simulink model "FOC_Control"  (R2024b)
settings: Solver=ode4  StartTime=0.0  StopTime=0.5  FixedStep=Ts/10  RelTol=1e-3
InitFcn:
  | foc_param;
values from neighbouring files (symbols this model uses):
  Iq_max = cast(Iq_max, FOC_dtype)    [foc_param.m]
  Ki_dq = make_foc_parameter(Ki_dq_val, FOC_dtype, 'Id/Iq current PI integral gain',     'V/(A*s)')    [foc_param.m]
  Ki_w = make_foc_parameter(Ki_w_val,  FOC_dtype, 'Speed PI integral gain',             'A/rad')    [foc_param.m]
  Kp_dq = make_foc_parameter(Kp_dq_val, FOC_dtype, 'Id/Iq current PI proportional gain', 'V/A')    [foc_param.m]
  Kp_w = make_foc_parameter(Kp_w_val,  FOC_dtype, 'Speed PI proportional gain',         'A/(rad/s)')    [foc_param.m]
  Spd_ref_tau = Kp_w_val/Ki_w_val    [foc_param.m]
  Ts = 1/20000    (= 5e-05)    [foc_param.m]
  Vmax = cast(Vmax,   FOC_dtype)    [foc_param.m]
undefined symbols (not defined in the file or in its folder): DiscIntNeverNeededParam
settings Model: Creator=BitCore  LastModifiedBy=BitCore
settings OptimizationCC: DefaultParameterBehavior=Inlined  EnhancedBackFolding=on  PassReuseOutputArgsAs=Individual arguments  ZeroExternalMemoryAtStartup=off  ZeroInternalMemoryAtStartup=off  OptimizeBlockOrder=speed  DifferentSizesBufferReuse=on  OptimizationCustomize=off  EfficientTunableParamExpr=on
settings DebuggingCC: ParameterTunabilityLossMsg=error
settings HardwareCC: ProdBitPerInt=16  ProdBitPerPointer=16  ProdBitPerSizeT=16  ProdBitPerPtrDiffT=16  ProdLargestAtomicFloat=None  ProdWordSize=16  ProdHWDeviceType=STMicroelectronics->ST10/Super10  TargetBitPerPointer=64  TargetBitPerSizeT=64  TargetBitPerPtrDiffT=64  TargetLongLongMode=on  TargetIntDivRoundTo=Zero  TargetEndianess=LittleEndian  TargetWordSize=64  TargetHWDeviceType=MATLAB Host  ProdEqTarget=off
settings SFSimCC: MATLABDynamicMemAlloc=off
settings RTWCC: Description=Embedded Coder (host-based shared library target)  SystemTargetFile=ert_shrlib.tlc  TemplateMakefile=ert_default_tmf
settings CodeAppCC: ForceParamTrailComments=on  IgnoreCustomStorageClasses=off  OperatorAnnotations=on  SimulinkDataObjDesc=on  SFDataObjDesc=on  InsertBlockDesc=on
settings STFCustomTargetCC: TargetLangStandard=C99 (ISO)  MultiwordLength=256  GenerateSampleERTMain=on  ParMdlRefBuildCompliant=on  CompOptLevelCompliant=on  CombineOutputUpdateFcns=on  ERTCustomFileBanners=on  SupportContinuousTime=off  SupportNonInlinedSFcns=off  RemoveResetFunc=on  MATLABClassNameForMDSCustomization=Simulink.SoftwareTarget.ERTCustomization  ModelStepFunctionPrototypeControlCompliant=on  UseToolchainInfoCompliant=on  SystemTargetFile=ert_shrlib.tlc
settings ERTTargetCC: TargetLangStandard=C99 (ISO)  GenerateSampleERTMain=on  ConcurrentExecutionCompliant=off  CPPClassGenCompliant=off  ERTCustomFileTemplate=example_file_process.tlc

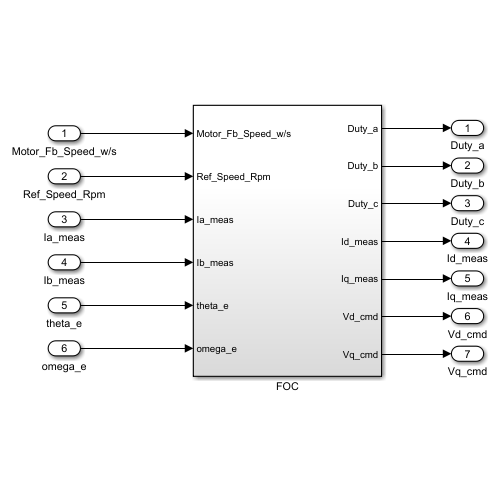
[thumbnail: Simulink's stored preview of the top-level diagram]
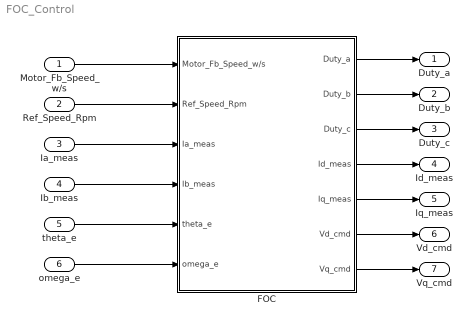
== system FOC_Control ==
  Motor_Fb_Speed_w/s : Inport
  Ref_Speed_Rpm : Inport  Port=2
  Ia_meas : Inport  Port=3
  Ib_meas : Inport  Port=4
  theta_e : Inport  Port=5
  omega_e : Inport  Port=6
  FOC : Subsystem
  Duty_a : Outport
  Duty_b : Outport  Port=2
  Duty_c : Outport  Port=3
  Id_meas : Outport  Port=4
  Iq_meas : Outport  Port=5
  Vd_cmd : Outport  Port=6
  Vq_cmd : Outport  Port=7
  wires:
  Motor_Fb_Speed_w/s/1 -> FOC/1(Motor_Fb_Speed_w/s)
  Ref_Speed_Rpm/1 -> FOC/2(Ref_Speed_Rpm)
  Ia_meas/1 -> FOC/3(Ia_meas)
  Ib_meas/1 -> FOC/4(Ib_meas)
  theta_e/1 -> FOC/5(theta_e)
  omega_e/1 -> FOC/6(omega_e)
  FOC/1(Duty_a) -> Duty_a/1
  FOC/2(Duty_b) -> Duty_b/1
  FOC/3(Duty_c) -> Duty_c/1
  FOC/4(Id_meas) -> Id_meas/1
  FOC/5(Iq_meas) -> Iq_meas/1
  FOC/6(Vd_cmd) -> Vd_cmd/1
  FOC/7(Vq_cmd) -> Vq_cmd/1

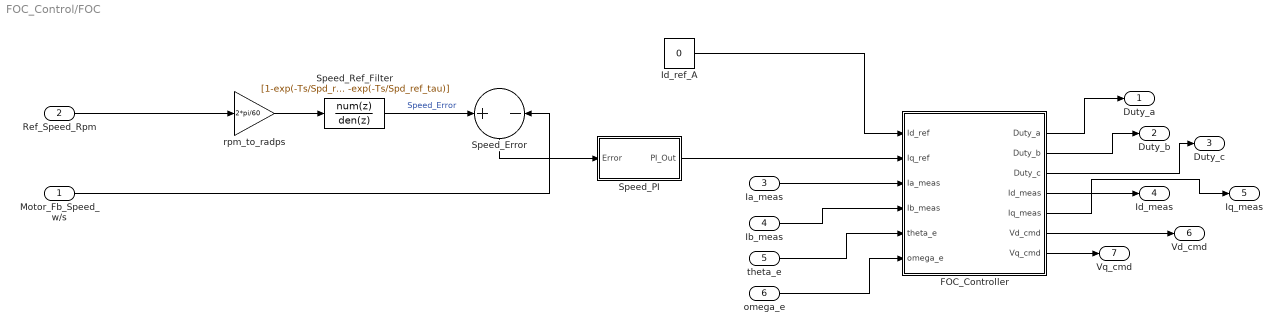
== system FOC_Control/FOC ==
  Motor_Fb_Speed_w/s : Inport
  Ref_Speed_Rpm : Inport  Port=2
  Ia_meas : Inport  Port=3
  Ib_meas : Inport  Port=4
  theta_e : Inport  Port=5
  omega_e : Inport  Port=6
  FOC_Controller : Subsystem
  Id_ref_A : Constant  Value=0
  Speed_Error : Sum  Inputs=+-
  Speed_PI : Subsystem
  Speed_Ref_Filter : DiscreteTransferFcn  Numerator=[1-exp(-Ts/Spd_ref_tau)]  Denominator=[1 -exp(-Ts/Spd_ref_tau)]  SampleTime=Ts
  rpm_to_radps : Gain  Gain=2*pi/60
  Duty_a : Outport
  Duty_b : Outport  Port=2
  Duty_c : Outport  Port=3
  Id_meas : Outport  Port=4
  Iq_meas : Outport  Port=5
  Vd_cmd : Outport  Port=6
  Vq_cmd : Outport  Port=7
  wires:
  Id_ref_A/1 -> FOC_Controller/1(Id_ref)
  Speed_Error/1 -> Speed_PI/1(Error)
  Ref_Speed_Rpm/1 -> rpm_to_radps/1
  Speed_Ref_Filter/1 -> Speed_Error/1  "Speed_Error"
  Speed_PI/1(PI_Out) -> FOC_Controller/2(Iq_ref)
  Motor_Fb_Speed_w/s/1 -> Speed_Error/2
  rpm_to_radps/1 -> Speed_Ref_Filter/1
  Ia_meas/1 -> FOC_Controller/3(Ia_meas)
  Ib_meas/1 -> FOC_Controller/4(Ib_meas)
  theta_e/1 -> FOC_Controller/5(theta_e)
  omega_e/1 -> FOC_Controller/6(omega_e)
  FOC_Controller/1(Duty_a) -> Duty_a/1
  FOC_Controller/2(Duty_b) -> Duty_b/1
  FOC_Controller/3(Duty_c) -> Duty_c/1
  FOC_Controller/4(Id_meas) -> Id_meas/1
  FOC_Controller/5(Iq_meas) -> Iq_meas/1
  FOC_Controller/6(Vd_cmd) -> Vd_cmd/1
  FOC_Controller/7(Vq_cmd) -> Vq_cmd/1

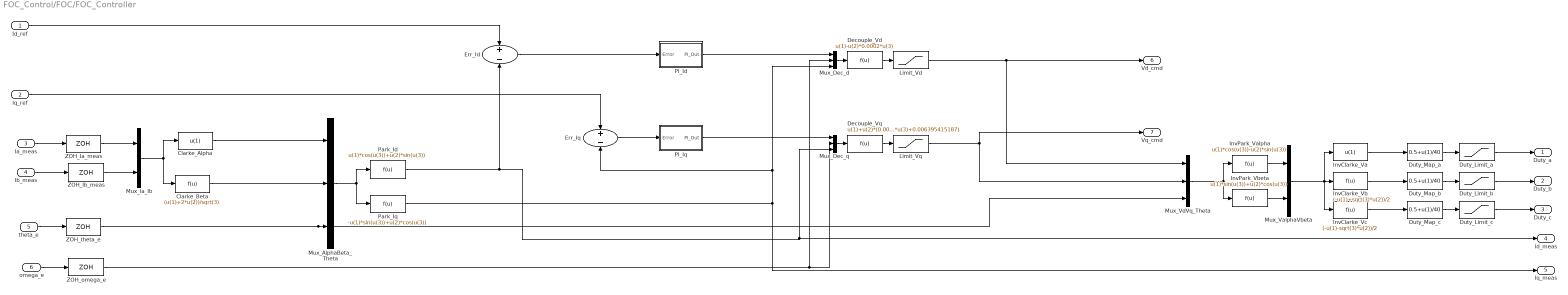
== system FOC_Control/FOC/FOC_Controller ==
  Id_ref : Inport
  Iq_ref : Inport  Port=2
  Ia_meas : Inport  Port=3
  Ib_meas : Inport  Port=4
  theta_e : Inport  Port=5
  omega_e : Inport  Port=6
  Clarke_Alpha : Fcn  Expr=u(1)
  Clarke_Beta : Fcn  Expr=(u(1)+2*u(2))/sqrt(3)
  Decouple_Vd : Fcn  Expr=u(1)-u(2)*0.0002*u(3)
  Decouple_Vq : Fcn  Expr=u(1)+u(2)*(0.0002*u(3)+0.006395415187)
  Duty_Limit_a : Saturate  UpperLimit=1  LowerLimit=0
  Duty_Limit_b : Saturate  UpperLimit=1  LowerLimit=0
  Duty_Limit_c : Saturate  UpperLimit=1  LowerLimit=0
  Duty_Map_a : Fcn  Expr=0.5+u(1)/40
  Duty_Map_b : Fcn  Expr=0.5+u(1)/40
  Duty_Map_c : Fcn  Expr=0.5+u(1)/40
  Err_Id : Sum  Inputs=+-
  Err_Iq : Sum  Inputs=+-
  InvClarke_Va : Fcn  Expr=u(1)
  InvClarke_Vb : Fcn  Expr=(-u(1)+sqrt(3)*u(2))/2
  InvClarke_Vc : Fcn  Expr=(-u(1)-sqrt(3)*u(2))/2
  InvPark_Valpha : Fcn  Expr=u(1)*cos(u(3))-u(2)*sin(u(3))
  InvPark_Vbeta : Fcn  Expr=u(1)*sin(u(3))+u(2)*cos(u(3))
  Limit_Vd : Saturate  UpperLimit=Vmax  LowerLimit=-Vmax
  Limit_Vq : Saturate  UpperLimit=Vmax  LowerLimit=-Vmax
  Mux_AlphaBeta_Theta : Mux  Inputs=3
  Mux_Dec_d : Mux  Inputs=3
  Mux_Dec_q : Mux  Inputs=3
  Mux_Ia_Ib : Mux  Inputs=2
  Mux_ValphaVbeta : Mux  Inputs=2
  Mux_VdVq_Theta : Mux  Inputs=3
  PI_Id : Subsystem
  PI_Iq : Subsystem
  Park_Id : Fcn  Expr=u(1)*cos(u(3))+u(2)*sin(u(3))
  Park_Iq : Fcn  Expr=-u(1)*sin(u(3))+u(2)*cos(u(3))
  ZOH_Ia_meas : ZeroOrderHold  SampleTime=Ts
  ZOH_Ib_meas : ZeroOrderHold  SampleTime=Ts
  ZOH_omega_e : ZeroOrderHold  SampleTime=Ts
  ZOH_theta_e : ZeroOrderHold  SampleTime=Ts
  Duty_a : Outport
  Duty_b : Outport  Port=2
  Duty_c : Outport  Port=3
  Id_meas : Outport  Port=4
  Iq_meas : Outport  Port=5
  Vd_cmd : Outport  Port=6
  Vq_cmd : Outport  Port=7
  wires:
  Ia_meas/1 -> ZOH_Ia_meas/1
  Ib_meas/1 -> ZOH_Ib_meas/1
  theta_e/1 -> ZOH_theta_e/1
  omega_e/1 -> ZOH_omega_e/1
  ZOH_Ia_meas/1 -> Mux_Ia_Ib/1
  ZOH_Ib_meas/1 -> Mux_Ia_Ib/2
  Mux_Ia_Ib/1 -> Clarke_Alpha/1, Clarke_Beta/1
  Clarke_Alpha/1 -> Mux_AlphaBeta_Theta/1
  Clarke_Beta/1 -> Mux_AlphaBeta_Theta/2
  ZOH_theta_e/1 -> Mux_VdVq_Theta/3, Mux_AlphaBeta_Theta/3
  Mux_AlphaBeta_Theta/1 -> Park_Id/1, Park_Iq/1
  Id_ref/1 -> Err_Id/1
  Park_Id/1 -> Id_meas/1, Mux_Dec_q/3, Err_Id/2
  Iq_ref/1 -> Err_Iq/1
  Park_Iq/1 -> Iq_meas/1, Mux_Dec_d/3, Err_Iq/2
  Err_Id/1 -> PI_Id/1(Error)
  Err_Iq/1 -> PI_Iq/1(Error)
  PI_Id/1(PI_Out) -> Mux_Dec_d/1
  ZOH_omega_e/1 -> Mux_Dec_d/2, Mux_Dec_q/2
  PI_Iq/1(PI_Out) -> Mux_Dec_q/1
  Mux_Dec_d/1 -> Decouple_Vd/1
  Mux_Dec_q/1 -> Decouple_Vq/1
  Decouple_Vd/1 -> Limit_Vd/1
  Decouple_Vq/1 -> Limit_Vq/1
  Limit_Vd/1 -> Vd_cmd/1, Mux_VdVq_Theta/1
  Limit_Vq/1 -> Vq_cmd/1, Mux_VdVq_Theta/2
  Mux_VdVq_Theta/1 -> InvPark_Vbeta/1, InvPark_Valpha/1
  InvPark_Valpha/1 -> Mux_ValphaVbeta/1
  InvPark_Vbeta/1 -> Mux_ValphaVbeta/2
  Mux_ValphaVbeta/1 -> InvClarke_Vc/1, InvClarke_Va/1, InvClarke_Vb/1
  InvClarke_Va/1 -> Duty_Map_a/1
  Duty_Map_a/1 -> Duty_Limit_a/1
  Duty_Limit_a/1 -> Duty_a/1
  InvClarke_Vb/1 -> Duty_Map_b/1
  Duty_Map_b/1 -> Duty_Limit_b/1
  Duty_Limit_b/1 -> Duty_b/1
  InvClarke_Vc/1 -> Duty_Map_c/1
  Duty_Map_c/1 -> Duty_Limit_c/1
  Duty_Limit_c/1 -> Duty_c/1

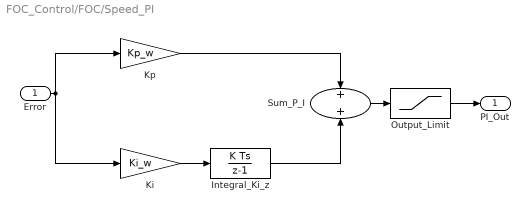
== system FOC_Control/FOC/Speed_PI ==
  Error : Inport
  Integral_Ki_z : DiscreteIntegrator  SampleTime=Ts  LimitOutput=on  UpperSaturationLimit=Iq_max  LowerSaturationLimit=-Iq_max  ICPrevOutput=DiscIntNeverNeededParam  ICPrevScaledInput=DiscIntNeverNeededParam
  Ki : Gain  Gain=Ki_w
  Kp : Gain  Gain=Kp_w
  Output_Limit : Saturate  UpperLimit=Iq_max  LowerLimit=-Iq_max
  Sum_P_I : Sum
  PI_Out : Outport
  wires:
  Error/1 -> Kp/1, Ki/1
  Ki/1 -> Integral_Ki_z/1
  Kp/1 -> Sum_P_I/1
  Integral_Ki_z/1 -> Sum_P_I/2
  Sum_P_I/1 -> Output_Limit/1
  Output_Limit/1 -> PI_Out/1

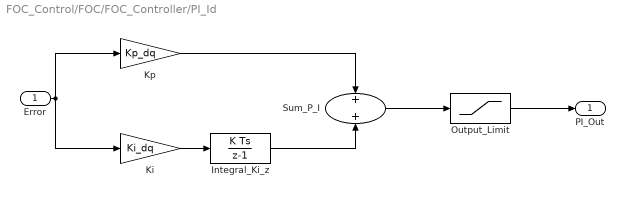
== system FOC_Control/FOC/FOC_Controller/PI_Id ==
  Error : Inport
  Integral_Ki_z : DiscreteIntegrator  SampleTime=Ts  LimitOutput=on  UpperSaturationLimit=Vmax  LowerSaturationLimit=-Vmax  ICPrevOutput=DiscIntNeverNeededParam  ICPrevScaledInput=DiscIntNeverNeededParam
  Ki : Gain  Gain=Ki_dq
  Kp : Gain  Gain=Kp_dq
  Output_Limit : Saturate  UpperLimit=Vmax  LowerLimit=-Vmax
  Sum_P_I : Sum
  PI_Out : Outport
  wires:
  Error/1 -> Kp/1, Ki/1
  Ki/1 -> Integral_Ki_z/1
  Kp/1 -> Sum_P_I/1
  Integral_Ki_z/1 -> Sum_P_I/2
  Sum_P_I/1 -> Output_Limit/1
  Output_Limit/1 -> PI_Out/1

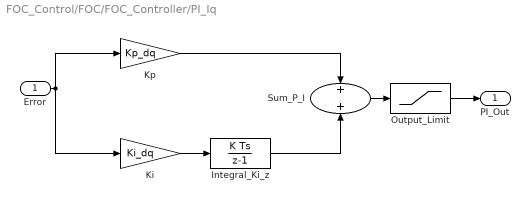
== system FOC_Control/FOC/FOC_Controller/PI_Iq ==
  Error : Inport
  Integral_Ki_z : DiscreteIntegrator  SampleTime=Ts  LimitOutput=on  UpperSaturationLimit=Vmax  LowerSaturationLimit=-Vmax  ICPrevOutput=DiscIntNeverNeededParam  ICPrevScaledInput=DiscIntNeverNeededParam
  Ki : Gain  Gain=Ki_dq
  Kp : Gain  Gain=Kp_dq
  Output_Limit : Saturate  UpperLimit=Vmax  LowerLimit=-Vmax
  Sum_P_I : Sum
  PI_Out : Outport
  wires:
  Error/1 -> Kp/1, Ki/1
  Ki/1 -> Integral_Ki_z/1
  Kp/1 -> Sum_P_I/1
  Integral_Ki_z/1 -> Sum_P_I/2
  Sum_P_I/1 -> Output_Limit/1
  Output_Limit/1 -> PI_Out/1
